simulink model "QD2_DroneStack_PID_2021a"  (R2022a)
settings: Solver=ode1  StartTime=0.0  StopTime=inf  FixedStep=1/1000  RelTol=1e-3  EnableMultiTasking=on
InitFcn:
  | Motor_Mapping_7_Inch
model workspace (MAT data in the model file):
  target_system = 1
values from neighbouring files (symbols this model uses):
  KT = [0.03616,0.117,-0.01215]    [Motor_Mapping_7_Inch.m]
  Motor_Matrix = [ 0.25   -1/(2*L_Roll)    1/(2*L_Pitch)    K_Tau/4;                  0.25   -1/(2*L_Roll)   -1/(2*L_Pitch)   -K_Tau/4;                  0.25    1/(2*L_Roll)    1/(2*L_Pitch)   -K_Tau/4;                  0.25    1/(2*L_Roll)   -1/(2*L_Pitch)    K_Tau/4]    [Motor_Mapping_7_Inch.m]
undefined symbols (not defined in the file or in its folder): _Commander, _QDrone2, _Stabilizer, datetime, HIL, lf, log_, m, n, qc_get_step_size, s, saved_data
libraries: quarc_library x94, simulink x27, simulink_extras x9
(part 1 of 4)
settings Model: DataTypeOverride=Double  MinMaxOverflowLogging=ForceOff  SimulationMode=external  ExtModeTrigDuration=10000  Creator=dmadill  LastModifiedBy=user
settings SolverCC: AlgebraicLoopSolver=TrustRegion  PositivePriorityOrder=on
settings DataIOCC: LimitDataPoints=on  SaveFormat=Array  ReturnWorkspaceOutputs=off
settings DebuggingCC: SolverPrmCheckMsg=warning  UnconnectedInputMsg=warning  UnconnectedOutputMsg=warning  UnconnectedLineMsg=warning  SFUnexpectedBacktrackingDiag=warning  SFNoUnconditionalDefaultTransitionDiag=warning  SFExecutionAtInitializationDiag=none  ArithmeticOperatorsInVariantConditions=warning
settings HardwareCC: ProdBitPerLong=64  ProdLargestAtomicInteger=LongLong  ProdLargestAtomicFloat=Double  ProdLongLongMode=on  ProdHWDeviceType=ARM Compatible->ARM 64-bit (LP64)
settings ModelReferenceCC: PropagateSignalLabelsOutOfModel=off
settings SFSimCC: SimUseLocalCustomCode=off  CustomCodeUndefinedFunction=UseInterfaceOnly
settings RTWCC: Description=QUARC Linux QDrone2 Target Using Toolchain  SystemTargetFile=quarc_linux_qdrone2.tlc  TemplateMakefile=quarc_default_tmf  RTWUseLocalCustomCode=off  Toolchain=QUARC linux_qdrone2 | gmake (64-bit Windows)  BuildConfiguration=Faster Runs  DLArmComputeVersion=19.05
settings CodeAppCC: StateflowObjectComments=on
settings STFCustomTargetCC: ConcurrentExecutionCompliant=on  UseToolchainInfoCompliant=on  SystemTargetFile=quarc_linux_qdrone2.tlc
settings GRTTargetCC: TargetLangStandard=C89/C90 (ANSI)  ParMdlRefBuildCompliant=off  CompOptLevelCompliant=off  CombineOutputUpdateFcns=off  MatFileLogging=off  CPPClassGenCompliant=off  GRTInterface=on  ExtMode=on  ExtModeMexFile=quarc_comm  ExtModeMexArgs='-w -d /tmp -uri %u -URI_Host tcpip://192.168.2.11:18001','tcpip://192.168.2.16:17001?retries=10'
settings ConfigComp: CovMetricSettings=dw  CovSaveCumulativeToWorkspaceVar=on  CovSaveSingleToWorkspaceVar=on  CovExternalEMLEnable=off  CovSFcnEnable=off

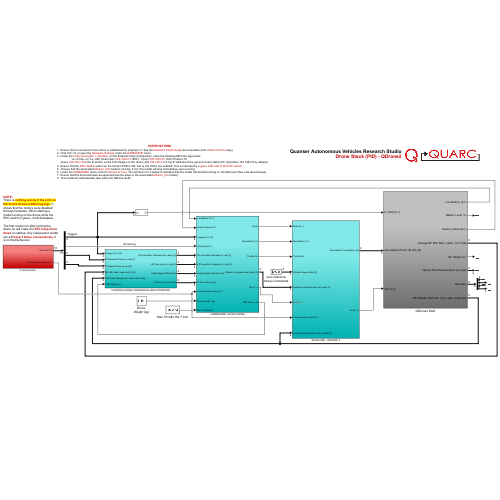
[thumbnail: Simulink's stored preview of the top-level diagram]
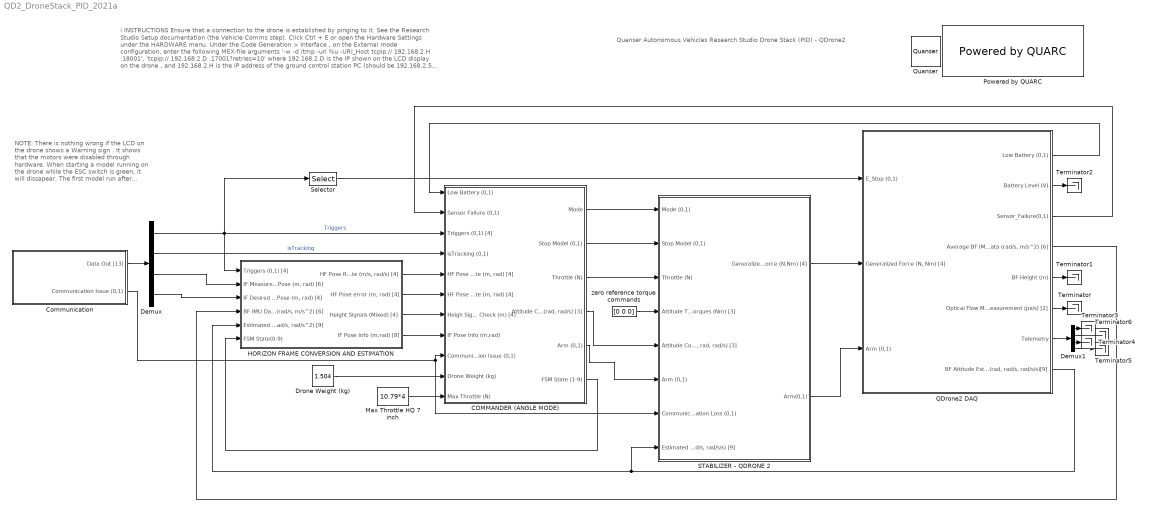
== system QD2_DroneStack_PID_2021a ==
  note: Quanser Autonomous Vehicles Research Studio
      | Drone Stack (PID) - QDrone2
  note: i
      | INSTRUCTIONS
      |
      | Ensure that a connection to the drone is established by pinging to it. See the Research Studio Setup documentation (the Vehicle Comms step).
      | Click Ctrl + E or open the Hardware Settings under the HARDWARE menu.
      | Under the Code Generation > Interface , on the External mode configuration, enter the following MEX-file arguments
      | '-w -d /tmp -uri %u -URI_Host tcpip:// 192.168.2.H :18001', 'tcpip:// 192.168.2.D :17001?retries=10'
      | where 192.168.2.D is the IP shown on the LCD display on the drone , and 192.168.2.H is the IP address of the ground control station PC (should be 192.168.2.5 by default).
      | Ensure that the ESC disable switch on the drone's PCB is ON, that is, the ESCs are enabled. This is indicated by a green LED next to the ESC switch .
      | . Ensure that the associated Mission_Ctrl model is running. If not, this model will stop immediately upon running.
      | Under the HARDWARE menu, click on Monitor & Tune . You will hear 3 to 5 beeps to indicates that the model has started running on the QDrone2 (See note about beeps).
      | Ensure that the drone behaves as expected (see the steps in the associated Mission_Ctrl model).
      | This model will automatically stop when the QDrone lands.
  note: NOTE:
      | There is nothing wrong if the LCD on the drone shows a Warning sign . It shows that the motors were disabled through hardware. When starting a model running on the drone while the ESC switch is green, it will dissapear.
      |
      | The first model run after turning the drone on will make the ESC beep three times on startup. Any subsequent model ran will beep 5 times consecutively. It is normal behaviour.
  COMMANDER (ANGLE MODE) : Subsystem
  Communication : Subsystem
  Demux : Demux  Outputs=[4 1 6 4]
  Demux1 : Demux
  Drone Weight (kg) : Constant  Value=1.504
  HORIZON FRAME CONVERSION AND ESTIMATION : Subsystem
  Max Throttle HQ 7 inch : Constant  Value=10.79*4
  Powered by QUARC : quarc_library/Logos/Powered by QUARC
  QDrone2 DAQ : Subsystem
  Quanser : quarc_library/Logos/Quanser
  STABILIZER - QDRONE 2 : Subsystem
  Selector : Selector  InputPortWidth=4  IndexOptions=Index vector (dialog)  Indices=[3]  OutputSizes=1
  Terminator{,1..6} (7 alike) : Terminator
  zero reference torque commands : Constant  Value=[0 0 0]
  wires:
  COMMANDER (ANGLE MODE)/2(Stop Model (0,1)) -> STABILIZER - QDRONE 2/2(Stop Model (0,1))
  zero reference torque commands/1 -> STABILIZER - QDRONE 2/4(Attitude Torques (Nm) [3])
  Communication/1(Data Out [13]) -> Demux/1
  QDrone2 DAQ/1(Low Battery (0,1)) -> COMMANDER (ANGLE MODE)/1(Low Battery (0,1))
  QDrone2 DAQ/3(Sensor_Failure(0,1)) -> COMMANDER (ANGLE MODE)/2(Sensor Failure (0,1))
  COMMANDER (ANGLE MODE)/4("Attitude Commands (rad, rad/s) [3]") -> STABILIZER - QDRONE 2/5("Attitude Commands (rad, rad, rad/s) [3]")
  COMMANDER (ANGLE MODE)/1(Mode) -> STABILIZER - QDRONE 2/1(Mode (0,1))
  QDrone2 DAQ/4("Average BF IMU Data (rad/s, m/s^2) [6]") -> HORIZON FRAME CONVERSION AND ESTIMATION/4("BF IMU Data (rad/s, m/s^2) [6]")
  Demux/4 -> HORIZON FRAME CONVERSION AND ESTIMATION/3("IF Desired Pose (m, rad) [4]")
  Demux/1 -> HORIZON FRAME CONVERSION AND ESTIMATION/1(Triggers (0,1) [4]), Selector/1, COMMANDER (ANGLE MODE)/3(Triggers (0,1) [4])  "Triggers"
  Demux/2 -> COMMANDER (ANGLE MODE)/4(isTracking (0,1))  "isTracking"
  Communication/2(Communication Issue (0,1)) -> COMMANDER (ANGLE MODE)/9(Communication Issue (0,1)), STABILIZER - QDRONE 2/7(Communication Loss (0,1))
  COMMANDER (ANGLE MODE)/6(FSM State (1-9)) -> HORIZON FRAME CONVERSION AND ESTIMATION/6(FSM State(0-9))
  HORIZON FRAME CONVERSION AND ESTIMATION/1("HF Pose Rate Estimate (m/s, rad/s) [4]") -> COMMANDER (ANGLE MODE)/5("HF Pose Rate Estimate (m, rad) [4]")
  HORIZON FRAME CONVERSION AND ESTIMATION/2("HF Pose error (m, rad) [4]") -> COMMANDER (ANGLE MODE)/6("HF Pose Error Estimate (m, rad) [4]")
  HORIZON FRAME CONVERSION AND ESTIMATION/3(Height Signals (Mixed) [4]) -> COMMANDER (ANGLE MODE)/7(Heigh Signals Check (m) [4])
  HORIZON FRAME CONVERSION AND ESTIMATION/4(IF Pose Info (m,rad) [8]) -> COMMANDER (ANGLE MODE)/8(IF Pose Info (m,rad))
  COMMANDER (ANGLE MODE)/3(Throttle (N)) -> STABILIZER - QDRONE 2/3(Throttle (N))
  QDrone2 DAQ/8("BF Attitude Estimate (rad, rad/s, rad/s/s)[9]") -> STABILIZER - QDRONE 2/8("Estimated Attitude (rad, rad/s, rad/s/s) [9]"), HORIZON FRAME CONVERSION AND ESTIMATION/5("Estimated Attitude (rad, rad/s, rad/s^2) [9]")
  STABILIZER - QDRONE 2/2(Arm(0,1)) -> QDrone2 DAQ/3(Arm (0,1))
  STABILIZER - QDRONE 2/1(Generalized Force (N,Nm) [4]) -> QDrone2 DAQ/2("Generalized Force (N, Nm) [4]")
  Drone Weight (kg)/1 -> COMMANDER (ANGLE MODE)/10(Drone Weight (kg))
  Max Throttle HQ 7 inch/1 -> COMMANDER (ANGLE MODE)/11(Max Throttle (N))
  Selector/1 -> QDrone2 DAQ/1(E_Stop (0,1))
  COMMANDER (ANGLE MODE)/5(Arm (0,1)) -> STABILIZER - QDRONE 2/6(Arm (0,1))
  QDrone2 DAQ/6(Optical Flow Measurement (px/s) [2]) -> Terminator/1
  QDrone2 DAQ/5("BF Height (m) ") -> Terminator1/1
  Demux/3 -> HORIZON FRAME CONVERSION AND ESTIMATION/2("IF Measured Pose (m, rad) [6]")
  QDrone2 DAQ/2(Battery Level (V)) -> Terminator2/1
  Demux1/1 -> Terminator3/1
  Demux1/3 -> Terminator4/1
  Demux1/2 -> Terminator6/1
  Demux1/4 -> Terminator5/1
  QDrone2 DAQ/7(Telemetry) -> Demux1/1

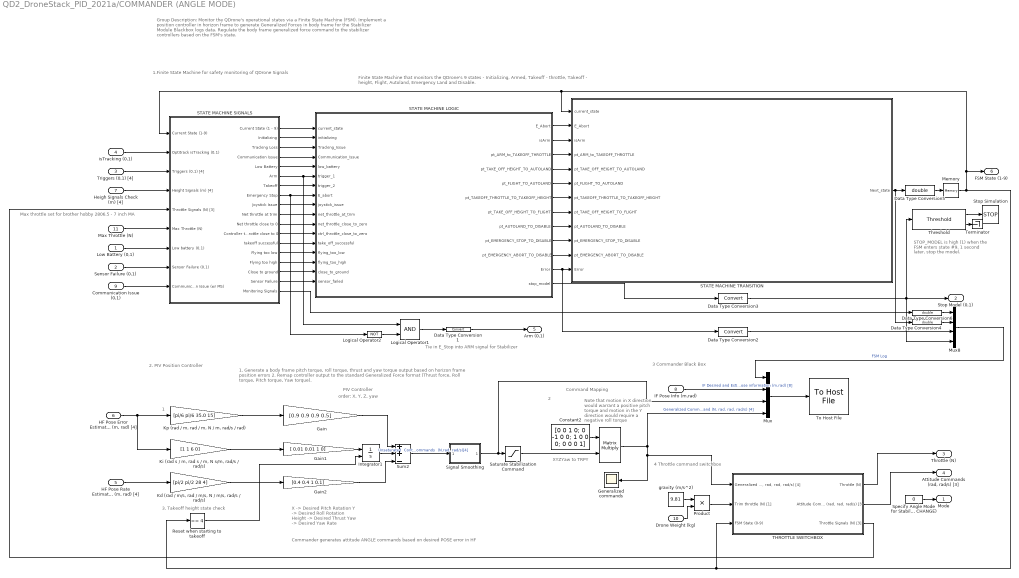
== system QD2_DroneStack_PID_2021a/COMMANDER (ANGLE MODE) ==
  note: 1.Finite State Machine for safety monitoring of QDrone Signals
  note: 2. PIV Position Controller
  note: Commander generates attitude ANGLE commands based on desired POSE error in HF
  note: 3 Commander Black Box
  note: 4 Throttle command switchbox
  note: Group Description:
      |
      | Monitor the QDrone's operational states via a Finite State Machine (FSM).
      | Implement a position controller in horizon frame to generate Generalized Forces in body frame for the Stabilizer Module
      | Blackbox logs data.
      | Regulate the body frame generalized force command to the stabilizer controllers based on the FSM's state.
  note: Note that motion in X direction would warrant a positive pitch torque
      | and motion in the Y direction would require a negative roll torque
  note: Command Mapping
  note: XYZYaw to TRPY
  note: 1
  note: 3. Takeoff height state check
  note: order: X, Y, Z, yaw
  note: 1. Generate a body frame pitch torque, roll torque, thrust and yaw torque output based on horizon frame position errors
      | 2. Remap controller output to the standard Generalized Force format (Thrust force, Roll torque, Pitch torque, Yaw torque).
  note: 2
  note: PIV Controller
  note: X -> Desired Pitch Rotation
      | Y -> Desired Roll Rotation
      | Height -> Desired Thrust
      | Yaw -> Desired Yaw Rate
  note: Finite State Machine that monitors the QDrone's 9 states - Initializing, Armed, Takeoff - throttle, Takeoff - height, Flight, Autoland, Emergency Land and Disable.
  note: Tie in E_Stop into ARM signal for Stabilizer
  note: STOP_MODEL is high (1) when
      | the FSM enters state #9.
      | 1 second later, stop the model.
  note: Max throttle set for brother hobby 2806.5 - 7 inch MA
  Low Battery (0,1) : Inport
  Sensor Failure (0,1) : Inport  Port=2
  Triggers (0,1) [4] : Inport  Port=3
  isTracking (0,1) : Inport  Port=4
  "HF Pose Rate Estimate (m, rad) [4]" : Inport  Port=5
  "HF Pose Error Estimate (m, rad) [4]" : Inport  Port=6
  Heigh Signals Check (m) [4] : Inport  Port=7
  IF Pose Info (m,rad) : Inport  Port=8
  Communication Issue (0,1) : Inport  Port=9
  Drone Weight (kg) : Inport  Port=10
  Max Throttle (N) : Inport  Port=11
  " " : Product  Multiplication=Matrix(*)
  Constant2 : Constant  Value=[0 0 1 0; 0 -1 0 0; 1 0 0 0; 0 0 0 1]
  Data Type Conversion1 : DataTypeConversion  SaturateOnIntegerOverflow=off  RndMeth=Floor
  Data Type Conversion2 : DataTypeConversion  SaturateOnIntegerOverflow=off  RndMeth=Floor
  Data Type Conversion3 : DataTypeConversion  SaturateOnIntegerOverflow=off  RndMeth=Floor
  Data Type Conversion4 : DataTypeConversion  OutDataTypeStr=double  SaturateOnIntegerOverflow=off  RndMeth=Floor
  Data Type Conversion5 : DataTypeConversion  OutDataTypeStr=double  SaturateOnIntegerOverflow=off  RndMeth=Floor
  Data Type Conversion6 : DataTypeConversion  OutDataTypeStr=double  SaturateOnIntegerOverflow=off  RndMeth=Floor
  Gain : Gain  Gain=[0.9 0.9 0.9 0.5]
  Gain1 : Gain  Gain=[ 0.01 0.01 1 0]
  Gain2 : Gain  Gain=[0.4 0.4 1 0.1]
  "Generalized commands " : Scope
  Integrator1 : Integrator  ExternalReset=rising  LimitOutput=on  UpperSaturationLimit=[0.26 0.33 15 0.05].*0.75  LowerSaturationLimit=[-0.26 -0.33 -15 -0.05].*0.75
  "Kd (rad / m/s, rad / m/s, N / m/s, rad/s / rad/s)" : Gain  Gain=[pi/2 pi/2 28 4]
  "Ki (rad s / m, rad s / m, N s/m, rad/s / rad/s)" : Gain  Gain=[1 1 6 0]
  "Kp (rad / m, rad / m, N / m, rad/s / rad)" : Gain  Gain=[pi/6 pi/6 35.0 15]
  Logical Operator1 : Logic  AllPortsSameDT=off  OutDataTypeStr=boolean
  Logical Operator2 : Logic  Operator=NOT  AllPortsSameDT=off  OutDataTypeStr=boolean
  Memory : Memory  InitialCondition=1
  Mux : Mux
  Mux8 : Mux  Inputs=[17 1 1 1]
  Product : Product
  Reset when starting to takeoff : simulink/Logic and Bit Operations/Compare To Constant  relop===  const=4  OutDataTypeStr=boolean
  STATE MACHINE LOGIC : MATLAB Function  TreatAsAtomicUnit=on
  STATE MACHINE SIGNALS : Subsystem
  STATE MACHINE TRANSITION : MATLAB Function  TreatAsAtomicUnit=on
  Saturate Stabilization Command : Saturate  UpperLimit=[pi/4 pi/4 35 100*pi/180]  LowerLimit=[-pi/4 -pi/4 -35 -100*pi/180]
  Signal Smoothing : Subsystem
  Specify Angle Mode for Stabilizer (DO NOT CHANGE) : Constant  Value=0
  Stop Simulation : Stop
  Sum2 : Sum  Inputs=++-
  "THROTTLE SWITCHBOX " : Subsystem
  Terminator : Terminator
  Threshold : quarc_library/Discontinuities/Threshold  operator=>=  param_src=Specify via dialog  threshold=0.5  duration=1
      settings: SourceProductName=QUARC Targets
  To Host File : quarc_library/Sinks/To Host/To Host File  file_name=saved_data/%m/log_%{regexprep(char(datetime),' ','_')}_Commander.mat  variable_name=commander_data  decimation=1  sample_time=-1  file_format=MAT-file v.5  options=No header or footer  append=off  final_file_name=saved_data/QD2_DroneStack_PID_2021a/log_20-Nov-2026_20-05-50_Commander.mat  bitrate=2000000
  gravity (m/s^2) : Constant  Value=9.81
  Mode : Outport  VectorParamsAs1DForOutWhenUnconnected=off
  Stop Model (0,1) : Outport  Port=2  VectorParamsAs1DForOutWhenUnconnected=off
  Throttle (N) : Outport  Port=3  VectorParamsAs1DForOutWhenUnconnected=off
  "Attitude Commands (rad, rad/s) [3]" : Outport  Port=4  VectorParamsAs1DForOutWhenUnconnected=off
  Arm (0,1) : Outport  Port=5  VectorParamsAs1DForOutWhenUnconnected=off
  FSM State (1-9) : Outport  Port=6  VectorParamsAs1DForOutWhenUnconnected=off
  wires:
  Mux8/1 -> Mux/1  "FSM Log"
  Specify Angle Mode for Stabilizer (DO NOT CHANGE)/1 -> Mode/1
  "THROTTLE SWITCHBOX "/1(Throttle (N)) -> Throttle (N)/1
  "THROTTLE SWITCHBOX "/3(Throttle Signals (N) [3]) -> STATE MACHINE SIGNALS/5(Throttle Signals (N) [3])
  Mux/1 -> To Host File/1
  IF Pose Info (m,rad)/1 -> Mux/2  "IF Desired and Estimated  pose information (m,rad) [8]"
  "THROTTLE SWITCHBOX "/2("Attitude Command (rad, rad, rad/s) [3]") -> "Attitude Commands (rad, rad/s) [3]"/1
  Sum2/1 -> Signal Smoothing/1("High Frequency Controller Commands (N,rad, rad/s)[4]")  "Unsaturated  Controller  Commands  (N,rad, rad/s)[4]"
  "Kd (rad / m/s, rad / m/s, N / m/s, rad/s / rad/s)"/1 -> Gain2/1
  "HF Pose Error Estimate (m, rad) [4]"/1 -> "Kp (rad / m, rad / m, N / m, rad/s / rad)"/1, "Ki (rad s / m, rad s / m, N s/m, rad/s / rad/s)"/1
  Saturate Stabilization Command/1 -> " "/2
  Constant2/1 -> " "/1
  Memory/1 -> "THROTTLE SWITCHBOX "/3(FSM State (0-9)), Reset when starting to takeoff/1, FSM State (1-9)/1, STATE MACHINE TRANSITION/1(current_state), STATE MACHINE SIGNALS/1(Current State (1-9))
  "HF Pose Rate Estimate (m, rad) [4]"/1 -> "Kd (rad / m/s, rad / m/s, N / m/s, rad/s / rad/s)"/1
  "Kp (rad / m, rad / m, N / m, rad/s / rad)"/1 -> Gain/1
  Integrator1/1 -> Sum2/2
  Reset when starting to takeoff/1 -> Integrator1/2
  " "/1 -> "Generalized commands "/1, "THROTTLE SWITCHBOX "/1("Generalized Command (N, rad, rad, rad/s) [4]"), Mux/4  "Generalized Command (N, rad, rad, rad/s) [4]"
  STATE MACHINE SIGNALS/1("Current State (1 - 9)  ") -> STATE MACHINE LOGIC/1(current_state)
  Threshold/1 -> Stop Simulation/1
  STATE MACHINE LOGIC/3(pt_ARM_to_TAKEOFF_THROTTLE) -> STATE MACHINE TRANSITION/4(pt_ARM_to_TAKEOFF_THROTTLE)
  Data Type Conversion5/1 -> Memory/1
  STATE MACHINE SIGNALS/5(Low Battery) -> STATE MACHINE LOGIC/5(low_battery)
  STATE MACHINE SIGNALS/8(Emergency Stop) -> Logical Operator2/1, STATE MACHINE LOGIC/8(E_abort)
  Data Type Conversion6/1 -> Mux8/1
  STATE MACHINE SIGNALS/11(Net throttle close to 0) -> STATE MACHINE LOGIC/11(net_throttle_close_to_zero)
  STATE MACHINE SIGNALS/16(Close to ground) -> STATE MACHINE LOGIC/16(close_to_ground)
  STATE MACHINE LOGIC/6(pt_TAKEOFF_THROTTLE_TO_TAKEOFF_HEIGHT) -> STATE MACHINE TRANSITION/7(pt_TAKEOFF_THROTTLE_TO_TAKEOFF_HEIGHT)
  STATE MACHINE LOGIC/12(stop_model) -> Data Type Conversion3/1
  STATE MACHINE SIGNALS/13(takeoff successful) -> STATE MACHINE LOGIC/13(take_off_successful)
  STATE MACHINE SIGNALS/7(Takeoff) -> STATE MACHINE LOGIC/7(trigger_2)
  STATE MACHINE TRANSITION/1(Next_state) -> Data Type Conversion5/1, Data Type Conversion4/1
  STATE MACHINE SIGNALS/4(Communication Issue) -> STATE MACHINE LOGIC/4(Communication_Issue)
  STATE MACHINE LOGIC/9(pt_EMERGENCY_STOP_TO_DISABLE) -> STATE MACHINE TRANSITION/10(pt_EMERGENCY_STOP_TO_DISABLE)
  STATE MACHINE LOGIC/5(pt_FLIGHT_TO_AUTOLAND) -> STATE MACHINE TRANSITION/6(pt_FLIGHT_TO_AUTOLAND)
  STATE MACHINE LOGIC/1(E_Abort) -> STATE MACHINE TRANSITION/2(E_Abort)
  STATE MACHINE SIGNALS/9("Joystick Issue ") -> STATE MACHINE LOGIC/9(joystick_issue)
  Data Type Conversion4/1 -> Mux8/2
  STATE MACHINE SIGNALS/12(Controller throttle close to 0) -> STATE MACHINE LOGIC/12(ctrl_throttle_close_to_zero)
  STATE MACHINE SIGNALS/14(Flying too low) -> STATE MACHINE LOGIC/14(flying_too_low)
  STATE MACHINE SIGNALS/15(Flying too high) -> STATE MACHINE LOGIC/15(flying_too_high)
  STATE MACHINE SIGNALS/10(Net throttle at trim) -> STATE MACHINE LOGIC/10(net_throttle_at_trim)
  STATE MACHINE SIGNALS/3(Tracking Loss) -> STATE MACHINE LOGIC/3(Tracking_Issue)
  STATE MACHINE SIGNALS/2(Initializing) -> STATE MACHINE LOGIC/2(initializing)
  Data Type Conversion1/1 -> Arm (0,1)/1
  STATE MACHINE LOGIC/2(isArm) -> STATE MACHINE TRANSITION/3(isArm)
  Data Type Conversion3/1 -> Threshold/1, Stop Model (0,1)/1, Mux8/4
  STATE MACHINE LOGIC/4(pt_TAKE_OFF_HEIGHT_TO_AUTOLAND) -> STATE MACHINE TRANSITION/5(pt_TAKE_OFF_HEIGHT_TO_AUTOLAND)
  Threshold/2 -> Terminator/1
  Data Type Conversion2/1 -> Mux8/3
  Logical Operator1/1 -> Data Type Conversion1/1
  STATE MACHINE SIGNALS/6(Arm) -> Logical Operator1/1, STATE MACHINE LOGIC/6(trigger_1)
  STATE MACHINE SIGNALS/18(Monitoring Signals) -> Data Type Conversion6/1
  STATE MACHINE LOGIC/7(pt_TAKE_OFF_HEIGHT_TO_FLIGHT) -> STATE MACHINE TRANSITION/8(pt_TAKE_OFF_HEIGHT_TO_FLIGHT)
  Logical Operator2/1 -> Logical Operator1/2
  STATE MACHINE LOGIC/10(pt_EMERGENCY_ABORT_TO_DISABLE) -> STATE MACHINE TRANSITION/11(pt_EMERGENCY_ABORT_TO_DISABLE)
  STATE MACHINE LOGIC/8(pt_AUTOLAND_TO_DISABLE) -> STATE MACHINE TRANSITION/9(pt_AUTOLAND_TO_DISABLE)
  STATE MACHINE SIGNALS/17("  Sensor Failure") -> STATE MACHINE LOGIC/17(sensor_failed)
  STATE MACHINE LOGIC/11(Error) -> Data Type Conversion2/1, STATE MACHINE TRANSITION/12(Error)
  Low Battery (0,1)/1 -> STATE MACHINE SIGNALS/7(Low battery (0,1))
  Sensor Failure (0,1)/1 -> STATE MACHINE SIGNALS/8(Sensor Failure (0,1))
  Communication Issue (0,1)/1 -> STATE MACHINE SIGNALS/9(Communication Issue (w/ MS))
  isTracking (0,1)/1 -> STATE MACHINE SIGNALS/2("Optitrack isTracking (0,1)  ")
  Triggers (0,1) [4]/1 -> STATE MACHINE SIGNALS/3(Triggers (0,1) [4])
  Heigh Signals Check (m) [4]/1 -> STATE MACHINE SIGNALS/4(Height Signals (m) [4])
  gravity (m/s^2)/1 -> Product/1
  Drone Weight (kg)/1 -> Product/2
  Product/1 -> "THROTTLE SWITCHBOX "/2(Trim throttle (N) [1])
  Max Throttle (N)/1 -> STATE MACHINE SIGNALS/6("Max Throttle (N) ")
  Gain/1 -> Sum2/1
  "Ki (rad s / m, rad s / m, N s/m, rad/s / rad/s)"/1 -> Gain1/1
  Gain1/1 -> Integrator1/1
  Gain2/1 -> Sum2/3
  Signal Smoothing/1("Smoothed Controller Commands (N,rad, rad/s)[4]") -> Saturate Stabilization Command/1, Mux/3

== system QD2_DroneStack_PID_2021a/Communication ==
  note: Argument (-URI_Host) is set at the MEX-file arguments found at Model Configuration Properties > Code Generation > Interface
      |
      | Format:
      | tcpip://192.168.2.H:18001
      | where H is the last digits of your ground station's IP address (use ipconfig in a command prompt to find it out).
  Constant : Constant
  Data Type Conversion : DataTypeConversion  SaturateOnIntegerOverflow=off  RndMeth=Floor
  Detect Communication Loss : Subsystem
  Memory : Memory  InheritSampleTime=on  LinearizeMemory=on  LinearizeAsDelay=on
  Model Argument : quarc_library/Sources/Signals/Model Argument  argument_name=URI_Host  has_value=on  data_type_mode=Specify via dialog  data_type=char  max_length=80  default_value=0  variable_size=off
      settings: AttributesFormatString=(-%<argument_name>)  SourceProductName=QUARC Targets
  Select Timestamp received and send back immediately (for calculating loopback time) : Selector  InputPortWidth=16  IndexOptions=Index vector (dialog)  Indices=[16]  OutputSizes=1
  Select the rest of the data : Selector  InputPortWidth=16  IndexOptions=Index vector (dialog)  Indices=[1:15]  OutputSizes=1
  Stream Client : quarc_library/Communications/Basic/Stream Client  uri_source=External input port  uri=tcpip://192.168.2.3:18669  send_buffer_size=1460  receive_buffer_size=1460  byte_order=little endian (Intel - LSB first)  optimization=Minimum latency  send_options=Send most recent data  receive_options=Receive most recent data  default_value=zeros(1,16)  sample_time=qc_get_step_size  active=off  implementation=Use blocking I/O in a separate thread  send_fifo_size=1000  receive_fifo_size=1000  send_priority=0  receive_priority=0  send_dimensions=off  receive_dimensions=off  max_dimensions=-1  data_type=Inherited via back propagation  type_expr=BusObject
  String Display : quarc_library/Strings/String Display  alignment=center  display_mode=Single line  sample_time=-1  use_new=off
      settings: SourceProductName=QUARC Targets
  Terminator1 : Terminator
  Terminator2 : Terminator
  Data Out [13] : Outport  VectorParamsAs1DForOutWhenUnconnected=off
  Communication Issue (0,1) : Outport  Port=2  VectorParamsAs1DForOutWhenUnconnected=off
  wires:
  Stream Client/5 -> Terminator2/1
  Model Argument/1 -> Stream Client/3, String Display/1
  Constant/1 -> Stream Client/2
  Stream Client/3 -> Terminator1/1
  Stream Client/4 -> Detect Communication Loss/3(Data Out), Data Type Conversion/1, Select the rest of the data/1
  Stream Client/1 -> Detect Communication Loss/1(State)
  Stream Client/2 -> Detect Communication Loss/2(Error)
  Detect Communication Loss/1(Communication Issue) -> Communication Issue (0,1)/1
  Select the rest of the data/1 -> Data Out [13]/1  "isTracking Triggers IF Measured Pose  IF Desired Pose"
  Select Timestamp received and send back immediately (for calculating loopback time)/1 -> Memory/1
  Memory/1 -> Stream Client/1
  Data Type Conversion/1 -> Select Timestamp received and send back immediately (for calculating loopback time)/1

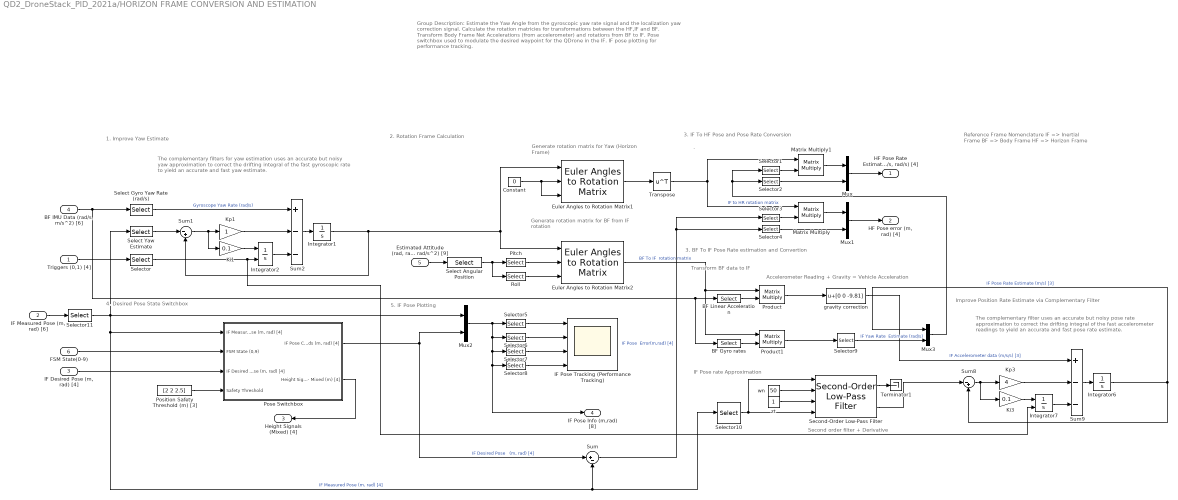
== system QD2_DroneStack_PID_2021a/HORIZON FRAME CONVERSION AND ESTIMATION ==
  note: 3. IF To HF Pose and Pose Rate Conversion
  note: IF Pose rate Approximation
  note: Transform BF data to IF
  note: 3. BF To IF Pose Rate estimation and Convertion
  note: 2. Rotation Frame Calculation
  note: .
  note: Reference Frame Nomenclature
      | IF => Inertial Frame
      | BF => Body Frame
      | HF => Horizon Frame
  note: Group Description:
      |
      | Estimate the Yaw Angle from the gyroscopic yaw rate signal and the localization yaw correction signal.
      | Calculate the rotation matricies for transformations between the HF,IF and BF.
      | Transform Body Frame Net Accelerations (from accelerometer) and rotations from BF to IF.
      | Pose switchbox used to modulate the desired waypoint for the QDrone in the IF.
      | IF pose plotting for performance tracking.
  note: 4. Desired Pose State Switchbox
  note: 5. IF Pose Plotting
  note: 1. Improve Yaw Estimate
  note: The complementary filters for yaw estimation uses an accurate but noisy yaw approximation to correct the drifting integral of the fast gyroscopic rate to yield an accurate and fast yaw estimate.
  note: Generate rotation matrix for Yaw
      | (Horizon Frame)
  note: Generate rotation matrix
      | for BF from IF rotation
  note: Accelerometer Reading + Gravity = Vehicle Acceleration
  note: The complementary filter uses an accurate but noisy pose rate approximation to correct the drifting integral of the fast accelerometer readings to yield an accurate and fast pose rate estimate.
  note: Second order filter + Derivative
  note: Improve Position Rate Estimate via Complementary Filter
  Triggers (0,1) [4] : Inport
  "IF Measured Pose (m, rad) [6]" : Inport  Port=2
  "IF Desired Pose (m, rad) [4]" : Inport  Port=3
  "BF IMU Data (rad/s, m/s^2) [6]" : Inport  Port=4
  "Estimated Attitude (rad, rad/s, rad/s^2) [9]" : Inport  Port=5
  FSM State(0-9) : Inport  Port=6
  BF Gyro rates : Selector  InputPortWidth=6  IndexOptions=Index vector (dialog)  Indices=[1:3]  OutputSizes=1
  BF Linear Acceleration : Selector  InputPortWidth=6  IndexOptions=Index vector (dialog)  Indices=[4:6]  OutputSizes=1
  Constant : Constant  Value=0
  Euler Angles to Rotation Matrix1 : quarc_library/Math Operations/Matrices/Euler Angles to Rotation Matrix  menu_order=Relative Z-Y-X
      settings: SourceProductName=QUARC Targets
  Euler Angles to Rotation Matrix2 : quarc_library/Math Operations/Matrices/Euler Angles to Rotation Matrix  menu_order=Relative Z-Y-X
      settings: SourceProductName=QUARC Targets
  IF Pose Tracking (Performance Tracking) : Scope  NumInputPorts=4
  Integrator1 : Integrator
  Integrator2 : Integrator  ExternalReset=rising
  Integrator6 : Integrator
  Integrator7 : Integrator  ExternalReset=rising
  Ki1 : Gain  Gain=0.1
  Ki3 : Gain  Gain=0.1
  Kp1 : Gain
  Kp3 : Gain  Gain=4
  Matrix Multiply : Product  Multiplication=Matrix(*)
  Matrix Multiply1 : Product  Multiplication=Matrix(*)
  Mux{,1..3} (4 alike) : Mux  Inputs=2
  Pitch : Selector  InputPortWidth=3  IndexOptions=Index vector (dialog)  Indices=[2]  OutputSizes=1
  Pose Switchbox : Subsystem
  Position Safety Threshold (m) [3] : Constant  Value=[2 2 2.5]
  Product : Product  Multiplication=Matrix(*)
  Product1 : Product  Multiplication=Matrix(*)
  Roll : Selector  InputPortWidth=3  IndexOptions=Index vector (dialog)  Indices=[1]  OutputSizes=1
  Second-Order Low-Pass Filter : quarc_library/Continuous/Second-Order Low-Pass Filter  params_source=External (input ports)  input_width=1  input_zeta=1  input_init=0
  Select Gyro Yaw Rate (rad/s) : Selector  InputPortWidth=6  IndexOptions=Index vector (dialog)  Indices=[3]  OutputSizes=1
  Select Angular Position : Selector  InputPortWidth=9  IndexOptions=Index vector (dialog)  Indices=[1:3]  OutputSizes=1
  Select Yaw Estimate : Selector  InputPortWidth=4  IndexOptions=Index vector (dialog)  Indices=4  OutputSizes=1
  Selector : Selector  InputPortWidth=4  IndexOptions=Index vector (dialog)  Indices=[2]  OutputSizes=1
  Selector1 : Selector  InputPortWidth=4  IndexOptions=Index vector (dialog)  Indices=[1:3]  OutputSizes=1
  Selector10 : Selector  InputPortWidth=4  IndexOptions=Index vector (dialog)  Indices=[1:3]  OutputSizes=1
  Selector11 : Selector  InputPortWidth=6  IndexOptions=Index vector (dialog)  Indices=[1:3,6]  OutputSizes=1
  Selector2 : Selector  InputPortWidth=4  IndexOptions=Index vector (dialog)  Indices=[4]  OutputSizes=1
  Selector3 : Selector  InputPortWidth=4  IndexOptions=Index vector (dialog)  Indices=[1:3]  OutputSizes=1
  Selector4 : Selector  InputPortWidth=4  IndexOptions=Index vector (dialog)  Indices=[4]  OutputSizes=1
  Selector5 : Selector  InputPortWidth=8  IndexOptions=Index vector (dialog)  Indices=[1 5]  OutputSizes=1
  Selector6 : Selector  InputPortWidth=8  IndexOptions=Index vector (dialog)  Indices=[2 6]  OutputSizes=1
  Selector7 : Selector  InputPortWidth=8  IndexOptions=Index vector (dialog)  Indices=[3 7]  OutputSizes=1
  Selector8 : Selector  InputPortWidth=8  IndexOptions=Index vector (dialog)  Indices=[4 8]  OutputSizes=1
  Selector9 : Selector  InputPortWidth=3  IndexOptions=Index vector (dialog)  Indices=[3]  OutputSizes=1
  Sum : Sum  Inputs=|+-
  Sum1 : Sum  Inputs=|-+
  Sum2 : Sum  Inputs=+--
  Sum8 : Sum  Inputs=|-+
  Sum9 : Sum  Inputs=+--
  Terminator1 : Terminator
  Transpose : Math  Operator=transpose  SignedPower=on
  gravity correction : Bias  Bias=[0 0 -9.81]  SaturateOnIntegerOverflow=off
  wn : Constant  Value=50
  zt : Constant
  "HF Pose Rate Estimate (m/s, rad/s) [4]" : Outport  VectorParamsAs1DForOutWhenUnconnected=off
  "HF Pose error (m, rad) [4]" : Outport  Port=2  VectorParamsAs1DForOutWhenUnconnected=off
  Height Signals (Mixed) [4] : Outport  Port=3  VectorParamsAs1DForOutWhenUnconnected=off
  IF Pose Info (m,rad) [8] : Outport  Port=4  VectorParamsAs1DForOutWhenUnconnected=off
  wires:
  Selector5/1 -> IF Pose Tracking (Performance Tracking)/1
  Selector7/1 -> IF Pose Tracking (Performance Tracking)/3
  Mux2/1 -> IF Pose Info (m,rad) [8]/1, Selector8/1, Selector7/1, Selector6/1, Selector5/1
  Selector6/1 -> IF Pose Tracking (Performance Tracking)/2
  Selector8/1 -> IF Pose Tracking (Performance Tracking)/4
  Selector4/1 -> Mux1/2
  Matrix Multiply/1 -> Mux1/1
  Selector3/1 -> Matrix Multiply/2
  Pose Switchbox/2(Height Signals - Mixed (m) [4]) -> Height Signals (Mixed) [4]/1
  Mux/1 -> "HF Pose Rate Estimate (m/s, rad/s) [4]"/1
  Selector2/1 -> Mux/2
  Selector1/1 -> Matrix Multiply1/2
  Matrix Multiply1/1 -> Mux/1
  Transpose/1 -> Matrix Multiply/1, Matrix Multiply1/1  "IF to HR rotation matrix"
  Mux3/1 -> Selector1/1, Selector2/1
  Mux1/1 -> "HF Pose error (m, rad) [4]"/1
  Sum/1 -> Selector3/1, Selector4/1  "IF Pose  Error(m,rad) [4]"
  FSM State(0-9)/1 -> Pose Switchbox/2(FSM State (0,9))
  Position Safety Threshold (m) [3]/1 -> Pose Switchbox/4(Safety Threshold)
  "BF IMU Data (rad/s, m/s^2) [6]"/1 -> Select Gyro Yaw Rate (rad/s)/1, BF Linear Acceleration/1, BF Gyro rates/1
  Select Gyro Yaw Rate (rad/s)/1 -> Sum2/1  "Gyroscope Yaw Rate (rad/s)"
  Triggers (0,1) [4]/1 -> Selector/1
  Select Angular Position/1 -> Roll/1, Pitch/1
  "IF Desired Pose (m, rad) [4]"/1 -> Pose Switchbox/3("IF Desired Pose (m, rad) [4]")
  BF Linear Acceleration/1 -> Product/2
  BF Gyro rates/1 -> Product1/2
  Integrator2/1 -> Sum2/3
  Select Yaw Estimate/1 -> Sum1/1
  Sum1/1 -> Ki1/1, Kp1/1
  Kp1/1 -> Sum2/2
  Sum2/1 -> Integrator1/1
  Ki1/1 -> Integrator2/1
  Roll/1 -> Euler Angles to Rotation Matrix2/3
  Pitch/1 -> Euler Angles to Rotation Matrix2/2
  Constant/1 -> Euler Angles to Rotation Matrix1/3, Euler Angles to Rotation Matrix1/2
  Integrator1/1 -> Euler Angles to Rotation Matrix2/1, Euler Angles to Rotation Matrix1/1, Sum1/2
  Euler Angles to Rotation Matrix1/1 -> Transpose/1
  Product1/1 -> Selector9/1
  Product/1 -> gravity correction/1
  Euler Angles to Rotation Matrix2/1 -> Product/1, Product1/1  "BF To IF  rotation matrix"
  Selector10/1 -> Second-Order Low-Pass Filter/4, Second-Order Low-Pass Filter/1
  Kp3/1 -> Sum9/2
  gravity correction/1 -> Sum9/1  "IF Accelerometer data (m/s/s) [3]"
  Second-Order Low-Pass Filter/2 -> Sum8/1
  Second-Order Low-Pass Filter/1 -> Terminator1/1
  zt/1 -> Second-Order Low-Pass Filter/3
  Ki3/1 -> Integrator7/1
  Sum8/1 -> Ki3/1, Kp3/1
  Integrator6/1 -> Sum8/2, Mux3/1  "IF Pose Rate Estimate (m/s) [3]"
  Sum9/1 -> Integrator6/1
  wn/1 -> Second-Order Low-Pass Filter/2
  Integrator7/1 -> Sum9/3
  Selector/1 -> Integrator7/2, Integrator2/2
  Selector9/1 -> Mux3/2  "IF Yaw Rate  Estimate (rad/s)"
  "IF Measured Pose (m, rad) [6]"/1 -> Selector11/1
  Pose Switchbox/1("IF Pose Commands (m, rad) [4]") -> Mux2/2, Sum/1  "IF Desired Pose   (m, rad) [4]"
  "Estimated Attitude (rad, rad/s, rad/s^2) [9]"/1 -> Select Angular Position/1
  Selector11/1 -> Mux2/1, Pose Switchbox/1("IF Measured Pose (m, rad) [4]"), Sum/2, Selector10/1, Select Yaw Estimate/1  "IF Measured Pose (m, rad) [4]"

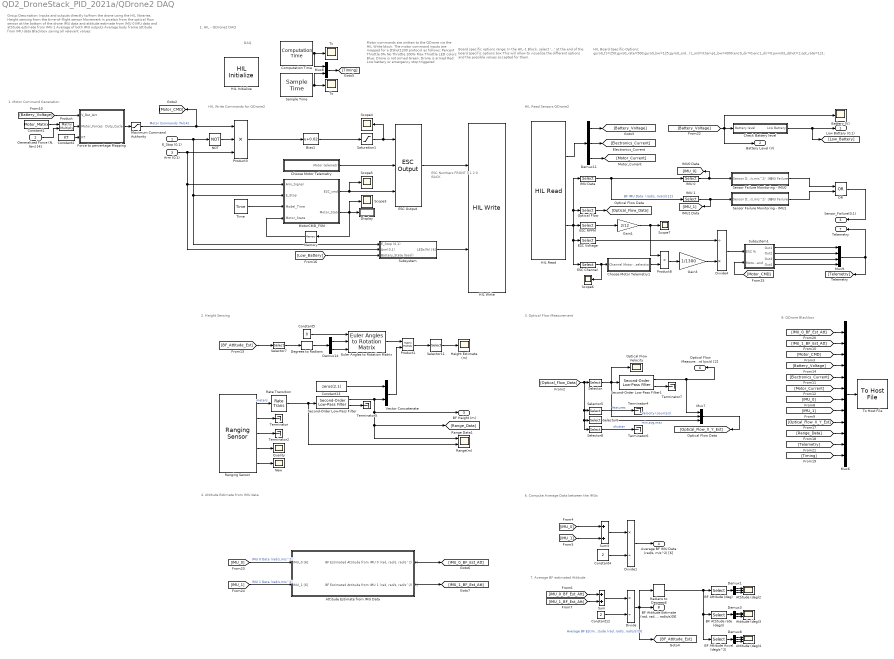
== system QD2_DroneStack_PID_2021a/QDrone2 DAQ ==
  note: 4. Attitude Estimate from IMU data
  note: 1. Motor Command Generation
  note: HIL Write Commands for QDrone2
  note: HIL Read Sensors QDrone2
  note: ESC Numbers
      |
      | FRONT
      | 3 1
      |
      | 2 0
      | BACK
  note: 1. HIL - QDrone2 DAQ
  note: Group Description:
      |
      | Inputs and outputs directly to/from the drone using the HIL libraries.
      | Height sensing from the time-of-flight sensor
      | Movement in pixels/s from the optical flow sensor at the bottom of the drone
      | IMU data and attitude estimate from IMU 0
      | IMU data and attitude estimate from IMU 1
      | Average of both IMU outputs
      | Average body frame attitude from IMU data
      | Blackbox saving all relevant values
  note: DAQ
  note: HIL Board Specific-Options:
      | gyro0_fs=250;gyro0_rate=500;gyro0_bw=125;gyro0_ord=3;accel0_fs=16;accel0_rate=1000;accel0_bw=400;accel0_ord=3;temp0_bw=4000;gyro1_fs=250;gyro1_rate=500;gyro1_bw=125;gyro1_ord=3;accel1_fs=16;accel1_rate=1000;accel1_bw=400;accel1_ord=3;temp1_bw=4000;enc0_dir=0;enc1_dir=0;pwm03_dshot=1;opt_rate=121;
  note: Motor commands are written to the QDrone via the HIL Write block. The motor command inputs are mapped for a DShot1200 protocol as follows:
      |
      | Percent Throttle
      | 0% No Throttle
      | 100% Max Throttle
      |
      | LED colors:
      | Blue: Drone is not armed
      | Green: Drone is armed
      | Red: Low battery or emergency stop triggered
  note: Board specific options range:
      |
      | In the HIL-1 Block,
      | select '...' at the end of the board specific options box
      | This will allow to visualize the different options
      | and the possible values accepted for them.
  note: 2. Height Sensing
  note: 8. QDrone Blackbox
  note: 6. Compute Average Data between the IMUs
  note: 7. Average BF estimated Attitude
  note: 3. Optical Flow Measurement
  E_Stop (0,1) : Inport
  "Generalized Force (N, Nm) [4]" : Inport  Port=2
  Arm (0,1) : Inport  Port=3
  Attitude (deg)2 : Scope  NumInputPorts=3
  Attitude (deg)3 : Scope  NumInputPorts=3
  Attitude (deg)4 : Scope  NumInputPorts=3
  Attitude Estimate from IMU Data : Subsystem
  BF Attitude (deg) : Selector  InputPortWidth=9  IndexOptions=Index vector (dialog)  Indices=[1:3]  OutputSizes=1
  BF Attitude Accel (deg/s^2) : Selector  InputPortWidth=9  IndexOptions=Index vector (dialog)  Indices=[7:9]  OutputSizes=1
  BF Attitude rate (deg/s) : Selector  InputPortWidth=9  IndexOptions=Index vector (dialog)  Indices=[4:6]  OutputSizes=1
  Battery (V) : Scope
  Bias1 : Bias  Bias=0.02  SaturateOnIntegerOverflow=off
  Check Battery level : Subsystem
  Choose Motor Telemetry : Subsystem
  Choose Motor Telemetry1 : Subsystem
  Computation Time : quarc_library/Sources/Time/Computation Time  sample_time=qc_get_step_size  use_model=on  use_cpu_time=off
  Constant1 : Constant  Value=Motor_Matrix  OutDataTypeStr=double
  Constant12 : Constant  Value=2
  Constant13 : Constant  Value=zeros(2,1)
  Constant2 : Constant  Value=KT  OutDataTypeStr=double
  Constant4 : Constant  Value=2
  Constant5 : Constant  Value=0
  Degrees to Radians : simulink_extras/Transformations/Degrees to Radians
  Demux{1,3,8,11} (4 alike) : Demux  Outputs=3
  Demux14 : Demux  Outputs=2
  Display : Display
  Divide : Product  Inputs=*/
  Divide1 : Product  Inputs=*/
  Divide4 : Product  Inputs=/*
  ESC Channel : Selector  InputPortWidth=22  IndexOptions=Index vector (dialog)  Indices=[22]  OutputSizes=1
  ESC Output : quarc_library/Data Acquisition/Generic/Transformations/ESC Output  protocol=DShot (raw)
      settings: AttributesFormatString=%<protocol>  SourceProductName=QUARC Targets
  ESC RPPM : Selector  InputPortWidth=22  IndexOptions=Index vector (dialog)  Indices=[20]  OutputSizes=1
  ESC Voltage : Selector  InputPortWidth=22  IndexOptions=Index vector (dialog)  Indices=[21]  OutputSizes=1
  Euler Angles to Rotation Matrix : quarc_library/Math Operations/Matrices/Euler Angles to Rotation Matrix  menu_order=Relative Z-X-Y
      settings: SourceProductName=QUARC Targets
  Force to percentage Mapping : MATLAB Function  TreatAsAtomicUnit=on
  Gain1 : Gain  Gain=2/12
  Gain3 : Gain  Gain=1/1300
  HIL Initialize : quarc_library/Data Acquisition/Generic/Configuration/HIL Initialize  object_name=HIL-1  board_type=qdrone2  board_number=0  board_options=gyro0_fs=250;gyro0_rate=500;gyro0_bw=125;gyro0_ord=3;accel0_fs=16;accel0_rate=1000;accel0_bw=400;accel0_ord=3;temp0_bw=4000;gyro1_fs=250;gyro1_rate=500;gyro1_bw=125;gyro1_ord=3;accel1_fs=16;accel1_rate=1000;accel1_bw=400;accel1_ord=3;temp1_bw=4000;enc0_dir=0;enc1_dir=0;pwm03_dshot=1;opt_rate=121;  exclusive=off  active=on  hardware_clocks=[]  clock_modes=[]  initial_clock_frequencies=[]  set_clock_params_at_start=off  set_clock_params_at_switch_in=off  set_clock_frequencies_at_start=off  set_clock_frequencies_at_switch_in=off  analog_input_channels=[0:4]  analog_input_configurations=[]  analog_input_maximums=[3.3]  analog_input_minimums=[0]  set_analog_input_params_at_start=off  set_analog_input_params_at_switch_in=off  analog_output_channels=[]  analog_output_maximums=[]  analog_output_minimums=[]  initial_analog_outputs=[]  final_analog_outputs=[]  watchdog_analog_outputs=[]  set_analog_output_params_at_start=off  set_analog_output_params_at_switch_in=off  set_analog_outputs_at_start=off  set_analog_outputs_at_switch_in=off  set_analog_outputs_at_terminate=off  set_analog_outputs_at_switch_out=off  set_analog_outputs_on_watchdog=off  digital_input_channels=[0:5]  digital_output_channels=[6:11]  digital_output_configuration=[]  initial_digital_outputs=[0]  final_digital_outputs=[0]  watchdog_digital_outputs=[0 0 0 0 0 0]  set_digital_output_params_at_start=off  set_digital_output_params_at_switch_in=off  set_digital_outputs_at_start=on  set_digital_outputs_at_switch_in=off  set_digital_outputs_at_terminate=on  set_digital_outputs_at_switch_out=off  set_digital_outputs_on_watchdog=off  encoder_channels=[0:1]  quadrature=[4]  encoder_filter_frequency=100e6/1  initial_encoder_counts=[0]  set_encoder_params_at_start=on  set_encoder_params_at_switch_in=off  set_encoder_counts_at_start=on  set_encoder_counts_at_switch_in=off  pwm_channels=[0:5]  pwm_modes=[6 6 6 6 0 0]  pwm_frequency=1.2e6  pwm_configuration=[0]  pwm_alignment=[0]  pwm_polarity=[1]  pwm_leading_deadband=[]  pwm_trailing_deadband=[]  initial_pwm_outputs=[0]  final_pwm_outputs=[0]  watchdog_pwm_outputs=[0]  set_pwm_params_at_start=on  set_pwm_params_at_switch_in=off  set_pwm_outputs_at_start=on  set_pwm_outputs_at_switch_in=off  set_pwm_outputs_at_terminate=on  set_pwm_outputs_at_switch_out=off  set_pwm_outputs_on_watchdog=off  other_output_channels=[]  initial_other_outputs=[0]  final_other_outputs=[0]  watchdog_other_outputs=[]  set_other_outputs_at_start=on  set_other_outputs_at_switch_in=off  set_other_outputs_at_terminate=on  set_other_outputs_at_switch_out=off  set_other_outputs_on_watchdog=off
  HIL Read : quarc_library/Data Acquisition/Generic/Immediate I//O/HIL Read  object_name=HIL-1  analog_channels=[3 1:2]  encoder_channels=[]  digital_channels=[]  other_channels=[3000:3002 4000:4002 3003:3005 4003:4005 17000:17006 17008:17009 17007]  sample_time=qc_get_step_size  active=on  vector_output=on  data_type_mode=Inherit via back propagation  encoder_data_type=double  digital_data_type=boolean
  HIL Write : quarc_library/Data Acquisition/Generic/Immediate I//O/HIL Write  object_name=HIL-1  analog_channels=[]  pwm_channels=[0:3]  digital_channels=[6:11]  other_channels=[]  sample_time=-1  active=off  vector_input=on
  Height Estimate (m) : Scope
  IMU 0 : Selector  InputPortWidth=12  IndexOptions=Index vector (dialog)  Indices=[1:6]  OutputSizes=1
  IMU 1 : Selector  InputPortWidth=12  IndexOptions=Index vector (dialog)  Indices=[7:12]  OutputSizes=1
  IMU Data : Selector  InputPortWidth=22  IndexOptions=Index vector (dialog)  Indices=[1:12]  OutputSizes=1
  "Maximum Command Authority " : Saturate  UpperLimit=[1 1 1 1]  LowerLimit=[0 0 0 0]
  Memory : Memory
  MotorCMD_FSM : MATLAB Function  TreatAsAtomicUnit=on
  Mux6 : Mux  Inputs=12
  Mux7 : Mux  Inputs=3
  Mux8 : Mux  Inputs=2
  Mux9 : Mux
  NOT : Logic  Operator=NOT  IconShape=distinctive  AllPortsSameDT=off  OutDataTypeStr=boolean
  New : Scope
  OR : Logic  Operator=OR  AllPortsSameDT=off  OutDataTypeStr=boolean
  Optical Flow : Selector  InputPortWidth=22  IndexOptions=Index vector (dialog)  Indices=[13:19]  OutputSizes=1
  Optical Flow Velocity : Scope
  Product : Product  Multiplication=Matrix(*)
  Product1 : Product  Multiplication=Matrix(*)
  Product3 : Product  Inputs=3
  Product8 : Product
  Quality : Scope
  Radians to Degrees6 : simulink_extras/Transformations/Radians to Degrees
  Range(m) : Scope  NumInputPorts=2
  Ranging Sensor : quarc_library/Devices/Third-Party/Sensors/Ranging Sensor  sensor_type=VL53L1X Time-of-flight  uri=i2c-cpu://localhost:0?address='0x29',baud='400000',memsize='512'  ranging_distance=Long  timing_budget=0.033  measurement_period=0.040  output_mode=Fixed-size output  samples_per_revolution=1300  max_distance=0.050  max_angle=5  sample_time=qc_get_step_size * ceil(1/121/ qc_get_step_size)  show_versions=off  active=on
      settings: SourceProductName=QUARC Targets
  Rate Transition : RateTransition
  Sample Time : quarc_library/Sources/Time/Sample Time  Priority=-99  sample_time=qc_get_step_size
  Saturation1 : Saturate  UpperLimit=1  LowerLimit=0
  Scope{3..7} (5 alike) : Scope
  Second-Order Low-Pass Filter : quarc_library/Continuous/Second-Order Low-Pass Filter  params_source=Internal (dialog parameters)  input_width=100  input_zeta=0.7  input_init=0
  Second-Order Low-Pass Filter1 : quarc_library/Continuous/Second-Order Low-Pass Filter  params_source=Internal (dialog parameters)  input_width=45  input_zeta=1.5  input_init=0
  Selector : Selector  InputPortWidth=7  IndexOptions=Index vector (dialog)  Indices=[1 2]  OutputSizes=1
  Selector11 : Selector  InputPortWidth=3  IndexOptions=Index vector (dialog)  Indices=[3]  OutputSizes=1
  Selector5 : Selector  InputPortWidth=7  IndexOptions=Index vector (dialog)  Indices=[3]  OutputSizes=1
  Selector6 : Selector  InputPortWidth=7  IndexOptions=Index vector (dialog)  Indices=[4 5 6]  OutputSizes=1
  Selector7 : Selector  InputPortWidth=9  IndexOptions=Index vector (dialog)  Indices=[1,2]  OutputSizes=1
  Selector8 : Selector  InputPortWidth=7  IndexOptions=Index vector (dialog)  Indices=[7]  OutputSizes=1
  Sensor Failure Monitoring - IMU0 : Subsystem
  Sensor Failure Monitoring - IMU1 : Subsystem
  Subsystem : Subsystem
  Subsystem1 : Subsystem
  Sum : Sum
  Sum3 : Sum
  Tc : Scope
  Terminator{,2,4..7} (6 alike) : Terminator
  Time : quarc_library/Sources/Time/Time  time_source=Wall clock  sample_time=qc_get_step_size
  To Host File : quarc_library/Sinks/To Host/To Host File  file_name=saved_data/%m/log_%{regexprep(char(datetime),' ','_')}_QDrone2.mat  variable_name=QDrone_data  decimation=1  sample_time=-1  file_format=MAT-file v.4  options=No header or footer  append=off  final_file_name=saved_data/QD2_DroneStack_PID_2021a/log_20-Nov-2026_20-05-50_QDrone2.mat  bitrate=2000000
  Ts : Scope
  Vector Concatenate : Concatenate
  Low Battery (0,1) : Outport
  Battery Level (V) : Outport  Port=2
  Sensor_Failure(0,1) : Outport  Port=3
  "Average BF IMU Data (rad/s, m/s^2) [6]" : Outport  Port=4
  "BF Height (m) " : Outport  Port=5
  Optical Flow Measurement (px/s) [2] : Outport  Port=6
  Telemetry : Outport  Port=7
  "BF Attitude Estimate (rad, rad/s, rad/s/s)[9]" : Outport  Port=8
  wires:
  Constant2/1 -> Force to percentage Mapping/3(KT)
  Constant1/1 -> Product/1
  "Generalized Force (N, Nm) [4]"/1 -> Product/2
  Product/1 -> Force to percentage Mapping/2(Motor_Forces)
  Force to percentage Mapping/1(Duty_Cycle) -> "Maximum Command Authority "/1
  "Maximum Command Authority "/1 -> Product3/1, [Motor_CMD]  "Motor Commands (%)[4]"
  [Battery_Voltage] -> Force to percentage Mapping/1(V_Bat_Act)
  Bias1/1 -> Saturation1/1
  ESC Voltage/1 -> Divide4/1
  IMU 0/1 -> Sensor Failure Monitoring - IMU0/1(Sensor Data (rad/s,m/s^2)  [6]), [IMU_0]
  OR/1 -> Sensor_Failure(0,1)/1
  Check Battery level/1(Low Battery) -> [Low_Battery], Low Battery (0,1)/1
  Optical Flow/1 -> [Optical_Flow_Data]
  IMU Data/1 -> IMU 0/1, IMU 1/1  "BF IMU Data  (rad/s, m/s/s)[12]"
  HIL Read/1 -> Demux11/1
  Gain1/1 -> Product8/1, Scope7/1
  NOT/1 -> Product3/2
  Memory/1 -> MotorCMD_FSM/4("Motor_State ")
  E_Stop (0,1)/1 -> Subsystem/1(E_Stop (0,1)), MotorCMD_FSM/2(E_Stop), NOT/1
  Subsystem/1(LEDs(%) [6]) -> HIL Write/2
  Demux11/2 -> [Electronics_Current]
  Sensor Failure Monitoring - IMU0/1(IMU Failure) -> OR/1
  ESC Output/1 -> HIL Write/1
  HIL Read/2 -> IMU Data/1, Optical Flow/1, ESC Voltage/1, ESC Channel/1, ESC RPPM/1
  [Battery_Voltage] -> Check Battery level/1(Battery level), Battery Level (V)/1, Battery (V)/1
  Demux11/3 -> [Motor_Current]
  IMU 1/1 -> [IMU_1], Sensor Failure Monitoring - IMU1/1(Sensor Data (rad/s,m/s^2)  [6])
  Choose Motor Telemetry1/1(Motor selection) -> Product8/2
  MotorCMD_FSM/2(Motor_State) -> Scope3/1, Display/1, Memory/1
  Gain3/1 -> Divide4/2
  Time/1 -> MotorCMD_FSM/3(Model_Time)
  Choose Motor Telemetry/1(Motor telemetry) -> ESC Output/2
  ESC Channel/1 -> Scope6/1, Choose Motor Telemetry1/1(Channel)
  Arm (0,1)/1 -> MotorCMD_FSM/1(Arm_Signal), Subsystem/2("Arm(0,1) "), Product3/3
  MotorCMD_FSM/1(ESC_cmd) -> Scope5/1, ESC Output/3
  Sensor Failure Monitoring - IMU1/1(IMU Failure) -> OR/2
  [Low_Battery] -> Subsystem/3(Battery_State (bool))
  ESC RPPM/1 -> Gain1/1
  Product8/1 -> Gain3/1
  Product3/1 -> Bias1/1
  Saturation1/1 -> ESC Output/1, Scope4/1
  Mux8/1 -> [Timing]
  Computation Time/1 -> Mux8/1, Tc/1
  Sample Time/1 -> Mux8/2, Ts/1
  Ranging Sensor/5 -> New/1
  [Range_Data] -> Mux6/10
  Selector5/1 -> Terminator4/1  "features"
  Mux7/1 -> [Optical_Flow_X_Y_Est]
  [Motor_CMD] -> Mux6/3
  Constant12/1 -> Divide/2
  Demux14/1 -> Euler Angles to Rotation Matrix/2
  Demux3/3 -> Attitude (deg)3/3
  Demux14/2 -> Euler Angles to Rotation Matrix/3
  [IMU_0_BF_Est_Att] -> Mux6/1
  [IMU_1_BF_Est_Att] -> Sum/2
  Mux9/1 -> [Telemetry], Telemetry/1
  [Optical_Flow_Data] -> Selector8/1, Selector6/1, Selector5/1, Selector/1
  BF Attitude Accel (deg/s^2)/1 -> Demux8/1
  Divide1/1 -> "Average BF IMU Data (rad/s, m/s^2) [6]"/1
  Subsystem1/4(Out4) -> Mux9/4
  [Timing] -> Mux6/12
  Selector6/1 -> Mux7/3  "min,avg,max"
  [Motor_CMD] -> Subsystem1/2(Motor command)
  [Telemetry] -> Mux6/11
  [IMU_1_BF_Est_Att] -> Mux6/2
  Constant13/1 -> Vector Concatenate/1
  [IMU_0] -> Sum3/1
  BF Attitude rate (deg/s)/1 -> Demux3/1
  Product1/1 -> Selector11/1
  [Motor_Current] -> Mux6/6
  Selector11/1 -> Height Estimate (m)/1
  Second-Order Low-Pass Filter/1 -> Vector Concatenate/2, [Range_Data], Range(m)/1, "BF Height (m) "/1
  Demux1/2 -> Attitude (deg)2/2
  Selector7/1 -> Degrees to Radians/1
  Constant5/1 -> Euler Angles to Rotation Matrix/1
  Second-Order Low-Pass Filter1/1 -> Mux7/1, Optical Flow Measurement (px/s) [2]/1
  Rate Transition/1 -> Range(m)/2, Second-Order Low-Pass Filter/1
  Subsystem1/3(Out3) -> Mux9/3
  Demux8/3 -> Attitude (deg)4/3
  Ranging Sensor/1 -> Rate Transition/1  "meters"
  Divide/1 -> "BF Attitude Estimate (rad, rad/s, rad/s/s)[9]"/1, [BF_Attitude_Est], Radians to Degrees6/1  "Average BF Estimated Attitude (rad, rad/s, rad/s/s)[9]"
  Degrees to Radians/1 -> Demux14/1
  Constant4/1 -> Divide1/2
  Euler Angles to Rotation Matrix/1 -> Product1/1
  [IMU_1] -> Sum3/2
  Demux1/3 -> Attitude (deg)2/3
  Demux8/2 -> Attitude (deg)4/2
  [IMU_1] -> Mux6/8
  [Optical_Flow_X_Y_Est] -> Mux6/9
  [BF_Attitude_Est] -> Selector7/1
  Ranging Sensor/4 -> Quality/1
  Subsystem1/1(Out1) -> Mux9/1
  Sum/1 -> Divide/1
  Vector Concatenate/1 -> Product1/2
  Demux3/1 -> Attitude (deg)3/1
  Selector8/1 -> Terminator6/1  "shutter"
  Radians to Degrees6/1 -> BF Attitude Accel (deg/s^2)/1, BF Attitude rate (deg/s)/1, BF Attitude (deg)/1
  Demux8/1 -> Attitude (deg)4/1
  Demux3/2 -> Attitude (deg)3/2
  Ranging Sensor/2 -> Terminator/1
  Ranging Sensor/3 -> Terminator2/1
  [IMU_0] -> Mux6/7
  Demux1/1 -> Attitude (deg)2/1
  [Battery_Voltage] -> Mux6/4
  Mux6/1 -> To Host File/1
  [Electronics_Current] -> Mux6/5
  [IMU_0_BF_Est_Att] -> Sum/1
  Divide4/1 -> Subsystem1/1(ESC %)
  BF Attitude (deg)/1 -> Demux1/1
  Sum3/1 -> Divide1/1
  Subsystem1/2(Out2) -> Mux9/2
  Selector/1 -> Second-Order Low-Pass Filter1/1, Mux7/2, Optical Flow Velocity/1  "Velocity (counts/s)"
  Demux11/1 -> [Battery_Voltage]
  Second-Order Low-Pass Filter/2 -> Terminator5/1
  Second-Order Low-Pass Filter1/2 -> Terminator7/1
  [IMU_0] -> Attitude Estimate from IMU Data/1(IMU_0 [6])  "IMU 0 Data (rad/s,m/s^2)"
  [IMU_1] -> Attitude Estimate from IMU Data/2(IMU_1 [6])  "IMU 1 Data (rad/s,m/s^2)"
  Attitude Estimate from IMU Data/1("BF Estimated Attitude from IMU 0 (rad, rad/s, rad/s^2) [9]") -> [IMU_0_BF_Est_Att]
  Attitude Estimate from IMU Data/2("BF Estimated Attitude from IMU 1 (rad, rad/s, rad/s^2) [9]") -> [IMU_1_BF_Est_Att]
